simulink model "TD3simu"  (R2024b)
settings: Solver=ode23t  StartTime=0.0  StopTime=5  RelTol=1e-3
values from neighbouring files (symbols this model uses):
  J = 0.5    [ABS.m]    (also in EBD.m; TD1_2_3.m = 0.2)
  L = 3    [EBD.m]    (also in TD1_2_3.m = 0.01216)
  p = 3    [TD1_2_3.m]
  phif = K/p    (= 0.3)    [TD1_2_3.m]
  R = 0.895    [TD1_2_3.m]
settings Model: Creator=E306-PC2  LastModifiedBy=julien.dbc

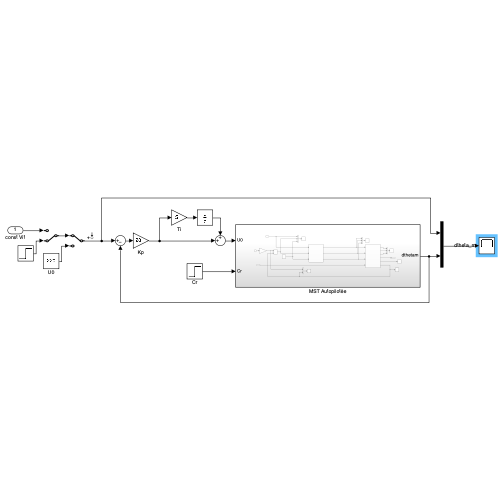
[thumbnail: Simulink's stored preview of the top-level diagram]
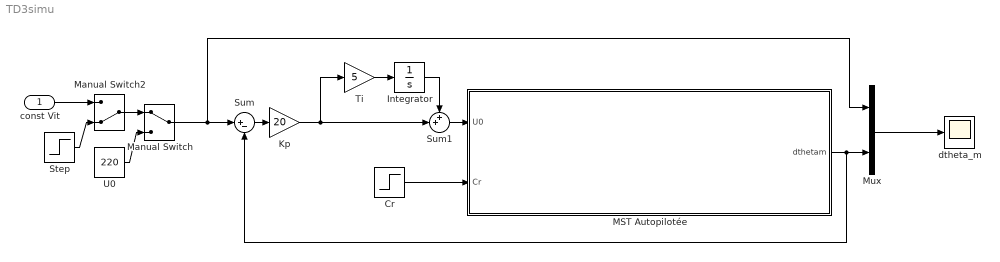
== system TD3simu ==
  const Vit : Inport
  Cr : Step  Time=3  After=100  SampleTime=0
  Integrator : Integrator
  Kp : Gain  Gain=20
  MST Autopilotée : Subsystem
  Manual Switch : ManualSwitch
  Manual Switch2 : ManualSwitch  CurrentSetting=0
  Mux : Mux  Inputs=2
  Step : Step  Time=0  After=10  SampleTime=0
  Sum : Sum  Inputs=|+-
  Sum1 : Sum  Inputs=++|
  Ti : Gain  Gain=5
  U0 : Constant  Value=220
  dtheta_m : Scope
  wires:
  U0/1 -> Manual Switch/2
  Manual Switch2/1 -> Manual Switch/1
  Step/1 -> Manual Switch2/2
  const Vit/1 -> Manual Switch2/1
  Manual Switch/1 -> Mux/1, Sum/1
  Sum/1 -> Kp/1
  Cr/1 -> MST Autopilotée/2(Cr)
  Kp/1 -> Sum1/2, Ti/1
  Sum1/1 -> MST Autopilotée/1(U0)
  Ti/1 -> Integrator/1
  Integrator/1 -> Sum1/1
  Mux/1 -> dtheta_m/1
  MST Autopilotée/1(dthetam) -> Sum/2, Mux/2

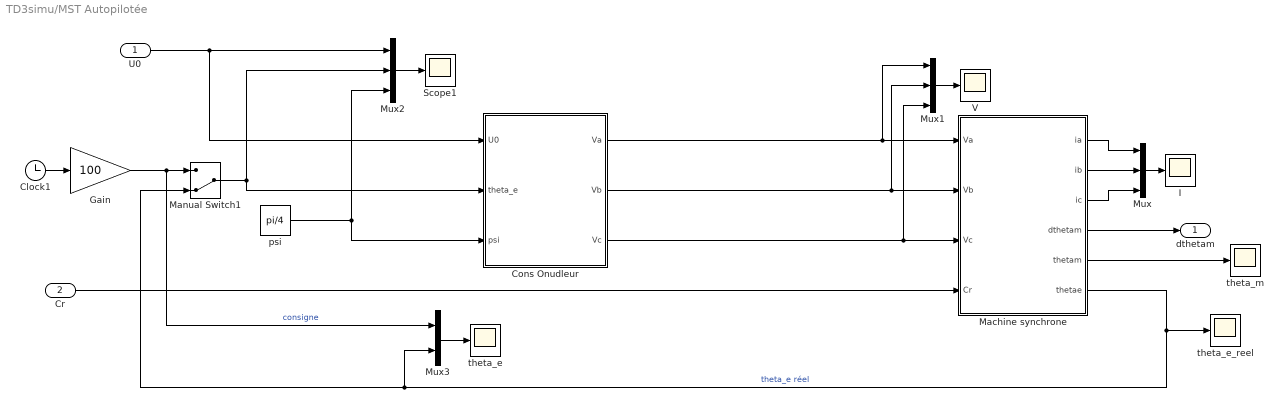
== system TD3simu/MST Autopilotée ==
  U0 : Inport
  Cr : Inport  Port=2
  Clock1 : Clock
      settings: Decimation=4
  Cons Onudleur : Subsystem
  Gain : Gain  Gain=100
  I : Scope
  Machine synchrone : Subsystem
  Manual Switch1 : ManualSwitch  CurrentSetting=0
  Mux : Mux  Inputs=3
  Mux1 : Mux  Inputs=3
  Mux2 : Mux  Inputs=3
  Mux3 : Mux  Inputs=2
  Scope1 : Scope
  V : Scope
  psi : Constant  Value=pi/4
  theta_e : Scope
  theta_e_reel : Scope
  theta_m : Scope
  dthetam : Outport
  wires:
  Machine synchrone/1(ia) -> Mux/1
  Mux/1 -> I/1
  Cons Onudleur/1(Va) -> Machine synchrone/1(Va), Mux1/1
  Machine synchrone/4(dthetam) -> dthetam/1
  Machine synchrone/2(ib) -> Mux/2
  Mux2/1 -> Scope1/1
  Machine synchrone/6(thetae) -> Manual Switch1/2, Mux3/2, theta_e_reel/1  "theta_e réel"
  Cons Onudleur/2(Vb) -> Mux1/2, Machine synchrone/2(Vb)
  Mux3/1 -> theta_e/1
  Machine synchrone/5(thetam) -> theta_m/1
  Clock1/1 -> Gain/1
  Manual Switch1/1 -> Cons Onudleur/2(theta_e), Mux2/2
  Cr/1 -> Machine synchrone/4(Cr)
  Machine synchrone/3(ic) -> Mux/3
  Cons Onudleur/3(Vc) -> Mux1/3, Machine synchrone/3(Vc)
  U0/1 -> Mux2/1, Cons Onudleur/1(U0)
  Mux1/1 -> V/1
  Gain/1 -> Manual Switch1/1, Mux3/1  "consigne"
  psi/1 -> Mux2/3, Cons Onudleur/3(psi)

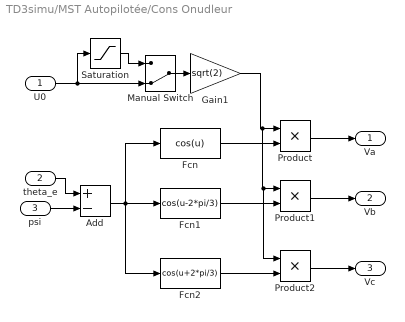
== system TD3simu/MST Autopilotée/Cons Onudleur ==
  U0 : Inport
  theta_e : Inport  Port=2
  psi : Inport  Port=3
  Add : Sum  Inputs=+-
  Fcn : Fcn  Expr=cos(u)
  Fcn1 : Fcn  Expr=cos(u-2*pi/3)
  Fcn2 : Fcn  Expr=cos(u+2*pi/3)
  Gain1 : Gain  Gain=sqrt(2)
  Manual Switch : ManualSwitch  CurrentSetting=0
  Product : Product
  Product1 : Product
  Product2 : Product
  Saturation : Saturate  UpperLimit=110  LowerLimit=-110
  Va : Outport
  Vb : Outport  Port=2
  Vc : Outport  Port=3
  wires:
  Product1/1 -> Vb/1
  Add/1 -> Fcn/1, Fcn2/1, Fcn1/1
  Fcn2/1 -> Product2/2
  Fcn/1 -> Product/2
  Gain1/1 -> Product2/1, Product1/1, Product/1
  Fcn1/1 -> Product1/2
  Product/1 -> Va/1
  Product2/1 -> Vc/1
  psi/1 -> Add/2
  theta_e/1 -> Add/1
  Manual Switch/1 -> Gain1/1
  U0/1 -> Saturation/1, Manual Switch/2
  Saturation/1 -> Manual Switch/1

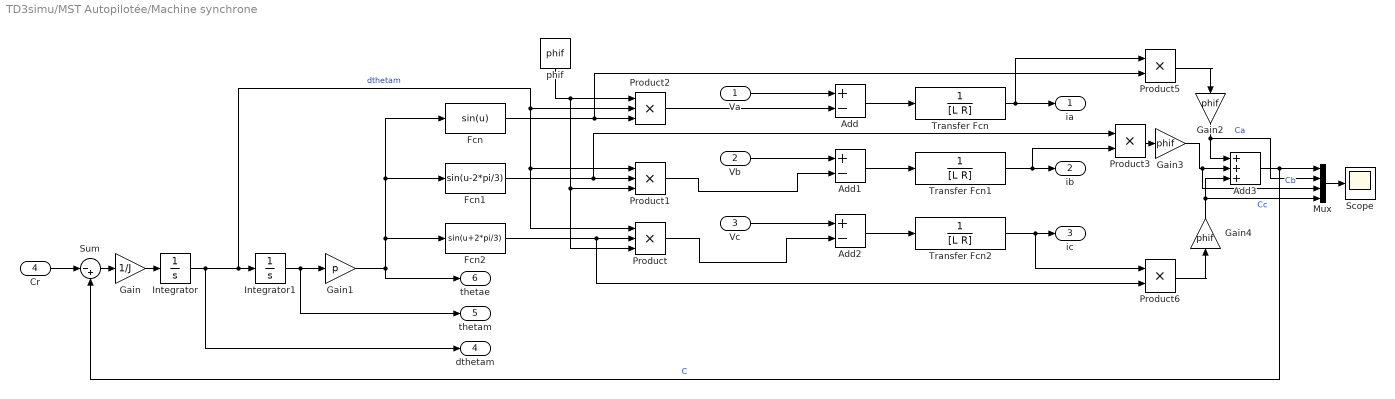
== system TD3simu/MST Autopilotée/Machine synchrone ==
  Va : Inport
  Vb : Inport  Port=2
  Vc : Inport  Port=3
  Cr : Inport  Port=4
  Add : Sum  Inputs=+-
  Add1 : Sum  Inputs=+-
  Add2 : Sum  Inputs=+-
  Add3 : Sum  Inputs=+++
  Fcn : Fcn  Expr=sin(u)
  Fcn1 : Fcn  Expr=sin(u-2*pi/3)
  Fcn2 : Fcn  Expr=sin(u+2*pi/3)
  Gain : Gain  Gain=1/J
  Gain1 : Gain  Gain=p
  Gain2 : Gain  Gain=phif
  Gain3 : Gain  Gain=phif
  Gain4 : Gain  Gain=phif
  Integrator : Integrator
  Integrator1 : Integrator
  Mux : Mux
  Product : Product  Inputs=3
  Product1 : Product  Inputs=3
  Product2 : Product  Inputs=3
  Product3 : Product
  Product5 : Product
  Product6 : Product
  Scope : Scope
  Sum : Sum  Inputs=|-+
  Transfer Fcn : TransferFcn  Denominator=[L R]
  Transfer Fcn1 : TransferFcn  Denominator=[L R]
  Transfer Fcn2 : TransferFcn  Denominator=[L R]
  phif : Constant  Value=phif
  ia : Outport
  ib : Outport  Port=2
  ic : Outport  Port=3
  dthetam : Outport  Port=4
  thetam : Outport  Port=5
  thetae : Outport  Port=6
  wires:
  Product2/1 -> Add/2
  Product6/1 -> Gain4/1
  Product5/1 -> Gain2/1
  Gain1/1 -> thetae/1, Fcn2/1, Fcn1/1, Fcn/1
  Fcn2/1 -> Product6/2, Product/2
  Va/1 -> Add/1
  Integrator1/1 -> thetam/1, Gain1/1
  Fcn1/1 -> Product3/1, Product1/2
  Integrator/1 -> dthetam/1, Product/1, Product1/1, Product2/2, Integrator1/1  "dthetam"
  Gain/1 -> Integrator/1
  phif/1 -> Product/3, Product1/3, Product2/1
  Fcn/1 -> Product5/2, Product2/3
  Add3/1 -> Mux/1, Sum/2  "C"
  Cr/1 -> Sum/1
  Sum/1 -> Gain/1
  Add/1 -> Transfer Fcn/1
  Transfer Fcn/1 -> Product5/1, ia/1
  Add1/1 -> Transfer Fcn1/1
  Product1/1 -> Add1/2
  Transfer Fcn1/1 -> Product3/2, ib/1
  Vb/1 -> Add1/1
  Add2/1 -> Transfer Fcn2/1
  Product/1 -> Add2/2
  Transfer Fcn2/1 -> Product6/1, ic/1
  Vc/1 -> Add2/1
  Mux/1 -> Scope/1
  Gain2/1 -> Mux/2, Add3/1  "Ca"
  Gain3/1 -> Mux/3, Add3/2  "Cb"
  Product3/1 -> Gain3/1
  Gain4/1 -> Mux/4, Add3/3  "Cc"
